simulink model "plant_3dof"  (R2026b)
settings: Solver=VariableStepAuto
undefined symbols (not defined in the file): p
libraries: simulink x1
settings Model: Creator=lorenzomonti  LastModifiedBy=lorenzomonti
settings ModelReferenceCC: ModelReferenceMinAlgLoopOccurrences=on

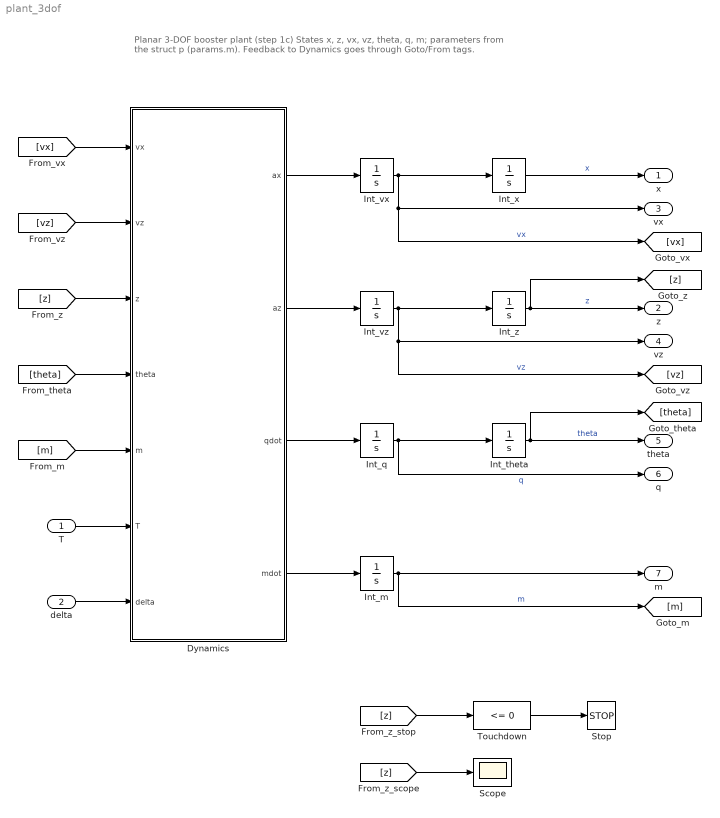
== system plant_3dof ==
  note: Planar 3-DOF booster plant (step 1c)
      | States x, z, vx, vz, theta, q, m; parameters from the struct p (params.m).
      | Feedback to Dynamics goes through Goto/From tags.
  T : Inport
  delta : Inport  Port=2
  Dynamics : MATLAB Function  TreatAsAtomicUnit=on
  Int_m : Integrator  InitialCondition=p.m0
  Int_q : Integrator  InitialCondition=p.q0
  Int_theta : Integrator  InitialCondition=p.theta0
  Int_vx : Integrator  InitialCondition=p.vx0
  Int_vz : Integrator  InitialCondition=p.vz0
  Int_x : Integrator  InitialCondition=p.x0
  Int_z : Integrator  InitialCondition=p.z0
  Scope : Scope
      settings: ActiveDisplayYMinimum=3080.5952098736093  ActiveDisplayYMaximum=5213.2671989029323
  Stop : Stop
  Touchdown : simulink/Logic and Bit Operations/Compare To Constant  relop=<=  const=0  OutDataTypeStr=boolean
  x : Outport
  z : Outport  Port=2
  vx : Outport  Port=3
  vz : Outport  Port=4
  theta : Outport  Port=5
  q : Outport  Port=6
  m : Outport  Port=7
  wires:
  [vx] -> Dynamics/1(vx)
  [vz] -> Dynamics/2(vz)
  [z] -> Dynamics/3(z)
  [theta] -> Dynamics/4(theta)
  [m] -> Dynamics/5(m)
  T/1 -> Dynamics/6(T)
  delta/1 -> Dynamics/7(delta)
  Dynamics/1(ax) -> Int_vx/1
  Dynamics/2(az) -> Int_vz/1
  Dynamics/3(qdot) -> Int_q/1
  Dynamics/4(mdot) -> Int_m/1
  Int_vx/1 -> vx/1, [vx], Int_x/1  "vx"
  Int_x/1 -> x/1  "x"
  Int_vz/1 -> vz/1, [vz], Int_z/1  "vz"
  Int_z/1 -> z/1, [z]  "z"
  Int_q/1 -> Int_theta/1, q/1  "q"
  Int_theta/1 -> theta/1, [theta]  "theta"
  Int_m/1 -> m/1, [m]  "m"
  [z] -> Touchdown/1
  Touchdown/1 -> Stop/1
  [z] -> Scope/1

== matlab function plant_3dof/Dynamics ==
  data: vx input; ax output; vz input; z input; theta input; m input; T input; delta input; az output; qdot output; mdot output; p parameter
function [ax, az, qdot, mdot] = dynamics(vx, vz, z, theta, m, T, delta, p)

if m <= p.mdry, T = 0; end

rho = p.rho0 * exp(-z/p.H);

V = sqrt((vx - p.wind)^2 + vz^2);

Dx = 0.5 * rho * p.CD * p.A * V * (vx - p.wind);
Dz = 0.5 * rho * p.CD * p.A * V * vz;

ax = (T * sin(theta + delta) - Dx)/m;
az = (T * cos(theta + delta) - Dz)/m - p.g;

qdot = - (T * p.l * sin(delta))/p.I;
mdot = - (T)/(p.Isp * p.g0);
